simulink model "esp32p4_foc"  (R2025b)
settings: Solver=FixedStepDiscrete  StartTime=0.0  StopTime=sim_end_s  FixedStep=Ts_plant  RelTol=1e-3
model workspace: external: MATLAB File esp32p4_foc_data.m (data not in the file)
values from neighbouring files (symbols this model uses):
  adc_bits = 12    [esp32p4_foc_data.m]
  adc_range_mV = 3100    [esp32p4_foc_data.m]
  alpha_w = 0.05    [esp32p4_foc_data.m]
  B_m = B_rotor + B_load    (= 1.07e-06)    [esp32p4_foc_data.m]
  b_u_mV = 1680    [esp32p4_foc_data.m]
  b_v_mV = 1680    [esp32p4_foc_data.m]
  ctrl_dt_max_s = 0.05    [esp32p4_foc_data.m]
  duty_mid = 0.5    [esp32p4_foc_data.m]
  enc_bits = 12    [esp32p4_foc_data.m]
  enc_dt_max_us = 20000    [esp32p4_foc_data.m]
  enc_dt_min_us = 100    [esp32p4_foc_data.m]
  enc_fail_decay = 0.9    [esp32p4_foc_data.m]
  enc_ok = 1    [esp32p4_foc_data.m]
  f_closed_max_Hz = 60    [esp32p4_foc_data.m]
  f_console_max_Hz = 80    [esp32p4_foc_data.m]
  I_console_max_mA = 1800    [esp32p4_foc_data.m]
  id_target_mA = 0    [esp32p4_foc_data.m]
  Imax = 200    [esp32p4_foc_data.m]
  J_m = J_rotor + J_load    (= 5e-07)    [esp32p4_foc_data.m]
  Ki_i = 8.0e-4    (= 0.0008)    [esp32p4_foc_data.m]
  Ki_w = 200    [esp32p4_foc_data.m]
  Kp_i = 2.5e-4    (= 0.00025)    [esp32p4_foc_data.m]
  Kp_w = 27    [esp32p4_foc_data.m]
  L_d = 2.58e-3    (= 0.00258)    [esp32p4_foc_data.m]
  L_q = L_d    (= 0.00258)    [esp32p4_foc_data.m]
  load_Nm = 0.002    [esp32p4_foc_data.m]
  mod_limit = 0.40    (= 0.4)    [esp32p4_foc_data.m]
  motor_x0 = [0; 0; 0; 0]    [esp32p4_foc_data.m]
  ocp_disable_s = 0.020    (= 0.02)    [esp32p4_foc_data.m]
  ocp_limit_mA = 1500    [esp32p4_foc_data.m]
  ocp_samples = 150    [esp32p4_foc_data.m]
  p_pairs = 7    [esp32p4_foc_data.m]
  psi_pm = Ke_LL_rms_per_krpm * sqrt(2/3) / (p_pairs * (1000*2*pi/60))    [esp32p4_foc_data.m]
  pwm_bits = 10    [esp32p4_foc_data.m]
  pwm_Hz = 20000    [esp32p4_foc_data.m]
  pwm_switching = 0    [esp32p4_foc_data.m]
  R_s = 18.76    [esp32p4_foc_data.m]
  R_shunt = 0.015    [esp32p4_foc_data.m]
  s_enc = 1    [esp32p4_foc_data.m]
  sense_gain = 50    [esp32p4_foc_data.m]
  sense_sign = -1    [esp32p4_foc_data.m]
  sense_wiring_sign = -1    [esp32p4_foc_data.m]
  start_Hz = 0    [esp32p4_foc_data.m]
  start_load_Nm = 0    [esp32p4_foc_data.m]
  step_load_s = 1.25    [esp32p4_foc_data.m]
  step_speed_s = 0.10    (= 0.1)    [esp32p4_foc_data.m]
  target_Hz = 8    [esp32p4_foc_data.m]
  theta_off = 0    [esp32p4_foc_data.m]
  torque_sign = 1    [esp32p4_foc_data.m]
  Ts_ctrl = 1e-3    (= 0.001)    [esp32p4_foc_data.m]
  Ts_plant = 1e-5    (= 1e-05)    [esp32p4_foc_data.m]
  unipolar_threshold_mV = 300    [esp32p4_foc_data.m]
  V_dc = 12    [esp32p4_foc_data.m]
Description:
  | ESP32-P4 M2: cascaded electrical speed and dq current control.
  | Firmware BassttElSevic/esp32p4-foc @ c20fad4. Starts calibrated in RUN.
  | Illustrative plant parameters are in the Model Workspace. Open the FOC subsystem to inspect the loops.
settings Model: Creator=29113  LastModifiedBy=29113
settings DataIOCC: SaveOutput=off  SaveTime=off

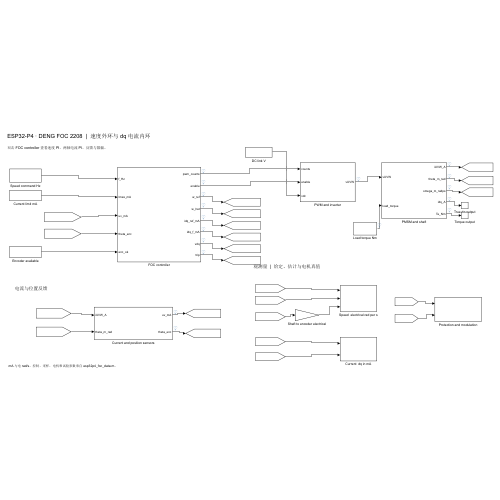
[thumbnail: Simulink's stored preview of the top-level diagram]
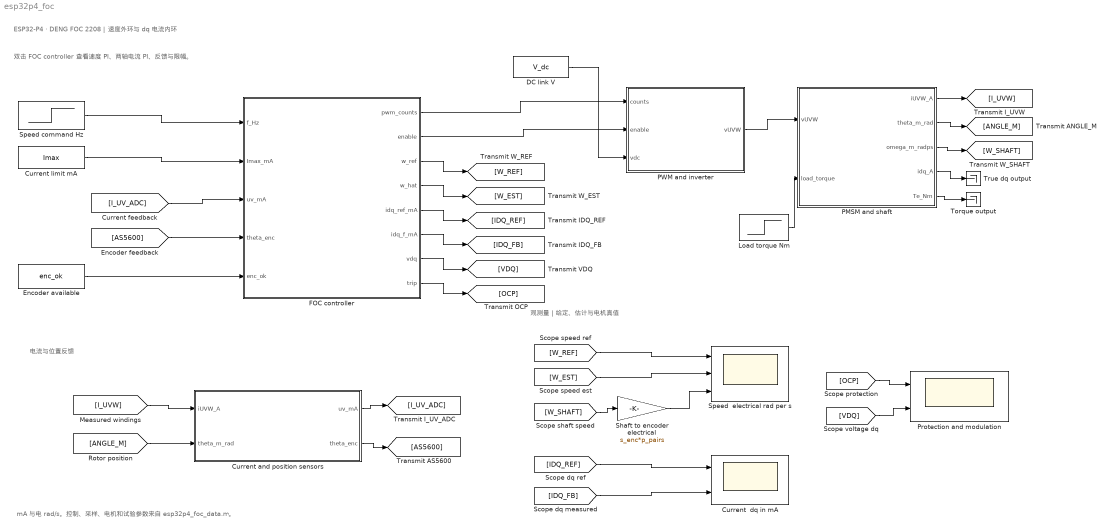
== system esp32p4_foc ==
  note: ESP32-P4 · DENG FOC 2208 | 速度外环与 dq 电流内环
  note: 双击 FOC controller 查看速度 PI、两轴电流 PI、反馈与限幅。
  note: 电流与位置反馈
  note: 观测量 | 给定、估计与电机真值
  note: mA 与电 rad/s。控制、采样、电机和试验参数来自 esp32p4_foc_data.m。
  Current  dq in mA : Scope  NumInputPorts=2
  Current and position sensors : Subsystem
  Current limit mA : Constant  Value=Imax  SampleTime=Ts_ctrl
  DC link V : Constant  Value=V_dc  SampleTime=Ts_plant
  Encoder available : Constant  Value=enc_ok  SampleTime=Ts_ctrl
  FOC controller : Subsystem
  Load torque Nm : Step  Time=step_load_s  Before=start_load_Nm  After=load_Nm  SampleTime=Ts_plant
  PMSM and shaft : Subsystem
  PWM and inverter : Subsystem
  Protection and modulation : Scope  NumInputPorts=2
  Shaft to encoder electrical : Gain  Gain=s_enc*p_pairs
  Speed  electrical rad per s : Scope  NumInputPorts=3
  Speed command Hz : Step  Time=step_speed_s  Before=start_Hz  After=target_Hz  SampleTime=Ts_ctrl
  Torque output : Terminator
  True dq output : Terminator
  wires:
  Speed command Hz/1 -> FOC controller/1(f_Hz)
  Current limit mA/1 -> FOC controller/2(Imax_mA)
  Encoder available/1 -> FOC controller/5(enc_ok)
  FOC controller/1(pwm_counts) -> PWM and inverter/1(counts)
  FOC controller/2(enable) -> PWM and inverter/2(enable)
  DC link V/1 -> PWM and inverter/3(vdc)
  PWM and inverter/1(vUVW) -> PMSM and shaft/1(vUVW)
  Load torque Nm/1 -> PMSM and shaft/2(load_torque)
  PMSM and shaft/1(iUVW_A) -> [I_UVW]
  PMSM and shaft/2(theta_m_rad) -> [ANGLE_M]
  [I_UVW] -> Current and position sensors/1(iUVW_A)
  [ANGLE_M] -> Current and position sensors/2(theta_m_rad)
  Current and position sensors/1(uv_mA) -> [I_UV_ADC]
  Current and position sensors/2(theta_enc) -> [AS5600]
  [I_UV_ADC] -> FOC controller/3(uv_mA)
  [AS5600] -> FOC controller/4(theta_enc)
  FOC controller/3(w_ref) -> [W_REF]
  FOC controller/4(w_hat) -> [W_EST]
  FOC controller/5(idq_ref_mA) -> [IDQ_REF]
  FOC controller/6(idq_f_mA) -> [IDQ_FB]
  FOC controller/7(vdq) -> [VDQ]
  FOC controller/8(trip) -> [OCP]
  PMSM and shaft/3(omega_m_radps) -> [W_SHAFT]
  PMSM and shaft/4(idq_A) -> True dq output/1
  PMSM and shaft/5(Te_Nm) -> Torque output/1
  [W_REF] -> Speed  electrical rad per s/1
  [W_EST] -> Speed  electrical rad per s/2
  [W_SHAFT] -> Shaft to encoder electrical/1
  Shaft to encoder electrical/1 -> Speed  electrical rad per s/3
  [IDQ_REF] -> Current  dq in mA/1
  [IDQ_FB] -> Current  dq in mA/2
  [OCP] -> Protection and modulation/1
  [VDQ] -> Protection and modulation/2

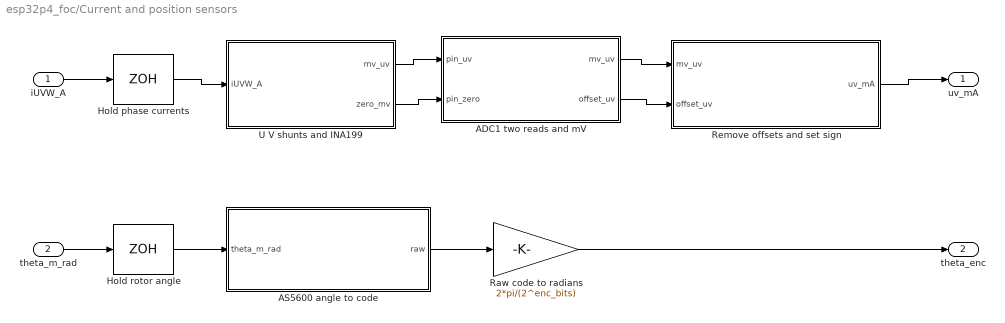
== system esp32p4_foc/Current and position sensors ==
  iUVW_A : Inport
  theta_m_rad : Inport  Port=2
  ADC1 two reads and mV : MATLAB Function  TreatAsAtomicUnit=on
  AS5600 angle to code : MATLAB Function  TreatAsAtomicUnit=on
  Hold phase currents : ZeroOrderHold  SampleTime=Ts_ctrl
  Hold rotor angle : ZeroOrderHold  SampleTime=Ts_ctrl
  Raw code to radians : Gain  Gain=2*pi/(2^enc_bits)
  Remove offsets and set sign : MATLAB Function  TreatAsAtomicUnit=on
  U V shunts and INA199 : MATLAB Function  TreatAsAtomicUnit=on
  uv_mA : Outport
  theta_enc : Outport  Port=2
  wires:
  iUVW_A/1 -> Hold phase currents/1
  Hold phase currents/1 -> U V shunts and INA199/1(iUVW_A)
  U V shunts and INA199/1(mv_uv) -> ADC1 two reads and mV/1(pin_uv)
  U V shunts and INA199/2(zero_mv) -> ADC1 two reads and mV/2(pin_zero)
  ADC1 two reads and mV/1(mv_uv) -> Remove offsets and set sign/1(mv_uv)
  ADC1 two reads and mV/2(offset_uv) -> Remove offsets and set sign/2(offset_uv)
  Remove offsets and set sign/1(uv_mA) -> uv_mA/1
  theta_m_rad/1 -> Hold rotor angle/1
  Hold rotor angle/1 -> AS5600 angle to code/1(theta_m_rad)
  AS5600 angle to code/1(raw) -> Raw code to radians/1
  Raw code to radians/1 -> theta_enc/1

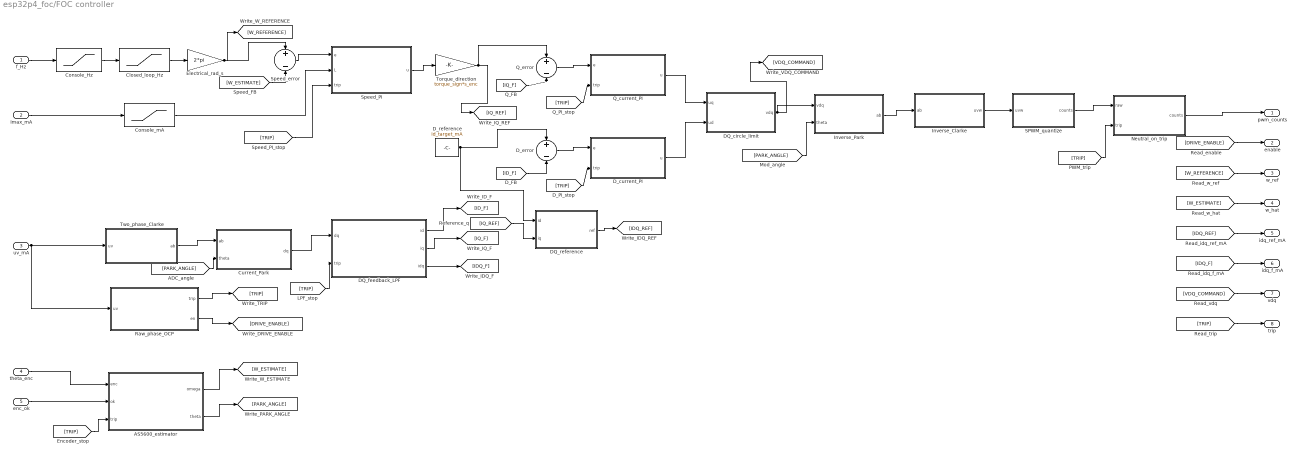
== system esp32p4_foc/FOC controller ==
  f_Hz : Inport
  Imax_mA : Inport  Port=2
  uv_mA : Inport  Port=3
  theta_enc : Inport  Port=4
  enc_ok : Inport  Port=5
  AS5600_estimator : MATLAB Function  TreatAsAtomicUnit=on
  Closed_loop_Hz : Saturate  UpperLimit=f_closed_max_Hz  LowerLimit=-f_closed_max_Hz
  Console_Hz : Saturate  UpperLimit=f_console_max_Hz  LowerLimit=-f_console_max_Hz
  Console_mA : Saturate  UpperLimit=I_console_max_mA  LowerLimit=-I_console_max_mA
  Current_Park : MATLAB Function  TreatAsAtomicUnit=on
  DQ_circle_limit : MATLAB Function  TreatAsAtomicUnit=on
  DQ_feedback_LPF : MATLAB Function  TreatAsAtomicUnit=on
  DQ_reference : MATLAB Function  TreatAsAtomicUnit=on
  D_current_PI : MATLAB Function  TreatAsAtomicUnit=on
  D_error : Sum  Inputs=+-
  D_reference : Constant  Value=id_target_mA
  Electrical_rad_s : Gain  Gain=2*pi
  Inverse_Clarke : MATLAB Function  TreatAsAtomicUnit=on
  Inverse_Park : MATLAB Function  TreatAsAtomicUnit=on
  Neutral_on_trip : MATLAB Function  TreatAsAtomicUnit=on
  Q_current_PI : MATLAB Function  TreatAsAtomicUnit=on
  Q_error : Sum  Inputs=+-
  Raw_phase_OCP : MATLAB Function  TreatAsAtomicUnit=on
  SPWM_quantize : MATLAB Function  TreatAsAtomicUnit=on
  Speed_PI : MATLAB Function  TreatAsAtomicUnit=on
  Speed_error : Sum  Inputs=+-
  Torque_direction : Gain  Gain=torque_sign*s_enc
  Two_phase_Clarke : MATLAB Function  TreatAsAtomicUnit=on
  pwm_counts : Outport
  enable : Outport  Port=2
  w_ref : Outport  Port=3
  w_hat : Outport  Port=4
  idq_ref_mA : Outport  Port=5
  idq_f_mA : Outport  Port=6
  vdq : Outport  Port=7
  trip : Outport  Port=8
  wires:
  Electrical_rad_s/1 -> [W_REFERENCE], Speed_error/1
  DQ_circle_limit/1(vdq) -> [VDQ_COMMAND], Inverse_Park/1(vdq)
  Torque_direction/1 -> [IQ_REF], Q_error/1
  DQ_feedback_LPF/1(id) -> [ID_F]
  DQ_feedback_LPF/2(iq) -> [IQ_F]
  DQ_feedback_LPF/3(idq) -> [IDQ_F]
  Raw_phase_OCP/1(trip) -> [TRIP]
  Raw_phase_OCP/2(en) -> [DRIVE_ENABLE]
  AS5600_estimator/1(omega) -> [W_ESTIMATE]
  AS5600_estimator/2(theta) -> [PARK_ANGLE]
  DQ_reference/1(ref) -> [IDQ_REF]
  [W_ESTIMATE] -> Speed_error/2
  [TRIP] -> Speed_PI/3(trip)
  [IQ_F] -> Q_error/2
  [ID_F] -> D_error/2
  [TRIP] -> Q_current_PI/2(trip)
  [TRIP] -> D_current_PI/2(trip)
  [PARK_ANGLE] -> Inverse_Park/2(theta)
  [TRIP] -> Neutral_on_trip/2(trip)
  [PARK_ANGLE] -> Current_Park/2(theta)
  [TRIP] -> DQ_feedback_LPF/2(trip)
  [TRIP] -> AS5600_estimator/3(trip)
  [IQ_REF] -> DQ_reference/2(iq)
  f_Hz/1 -> Console_Hz/1
  Console_Hz/1 -> Closed_loop_Hz/1
  Closed_loop_Hz/1 -> Electrical_rad_s/1
  Speed_error/1 -> Speed_PI/1(e)
  Imax_mA/1 -> Console_mA/1
  Console_mA/1 -> Speed_PI/2(L)
  Speed_PI/1(u) -> Torque_direction/1
  Q_error/1 -> Q_current_PI/1(e)
  D_reference/1 -> D_error/1, DQ_reference/1(id)
  D_error/1 -> D_current_PI/1(e)
  Q_current_PI/1(u) -> DQ_circle_limit/1(uq)
  D_current_PI/1(u) -> DQ_circle_limit/2(ud)
  Inverse_Park/1(ab) -> Inverse_Clarke/1(ab)
  Inverse_Clarke/1(uvw) -> SPWM_quantize/1(uvw)
  SPWM_quantize/1(counts) -> Neutral_on_trip/1(raw)
  uv_mA/1 -> Two_phase_Clarke/1(uv), Raw_phase_OCP/1(uv)
  Two_phase_Clarke/1(ab) -> Current_Park/1(ab)
  Current_Park/1(dq) -> DQ_feedback_LPF/1(dq)
  theta_enc/1 -> AS5600_estimator/1(enc)
  enc_ok/1 -> AS5600_estimator/2(ok)
  Neutral_on_trip/1(counts) -> pwm_counts/1
  [DRIVE_ENABLE] -> enable/1
  [W_REFERENCE] -> w_ref/1
  [W_ESTIMATE] -> w_hat/1
  [IDQ_REF] -> idq_ref_mA/1
  [IDQ_F] -> idq_f_mA/1
  [VDQ_COMMAND] -> vdq/1
  [TRIP] -> trip/1

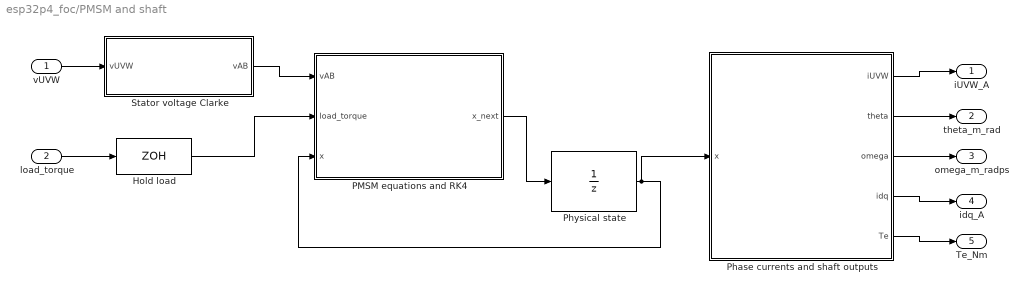
== system esp32p4_foc/PMSM and shaft ==
  vUVW : Inport
  load_torque : Inport  Port=2
  Hold load : ZeroOrderHold  SampleTime=Ts_plant
  PMSM equations and RK4 : MATLAB Function  TreatAsAtomicUnit=on
  Phase currents and shaft outputs : MATLAB Function  TreatAsAtomicUnit=on
  Physical state : UnitDelay  InitialCondition=motor_x0  SampleTime=Ts_plant  HasFrameUpgradeWarning=on
  Stator voltage Clarke : MATLAB Function  TreatAsAtomicUnit=on
  iUVW_A : Outport
  theta_m_rad : Outport  Port=2
  omega_m_radps : Outport  Port=3
  idq_A : Outport  Port=4
  Te_Nm : Outport  Port=5
  wires:
  Phase currents and shaft outputs/1(iUVW) -> iUVW_A/1
  Phase currents and shaft outputs/2(theta) -> theta_m_rad/1
  Phase currents and shaft outputs/3(omega) -> omega_m_radps/1
  Phase currents and shaft outputs/4(idq) -> idq_A/1
  Phase currents and shaft outputs/5(Te) -> Te_Nm/1
  vUVW/1 -> Stator voltage Clarke/1(vUVW)
  Stator voltage Clarke/1(vAB) -> PMSM equations and RK4/1(vAB)
  load_torque/1 -> Hold load/1
  Hold load/1 -> PMSM equations and RK4/2(load_torque)
  Physical state/1 -> PMSM equations and RK4/3(x), Phase currents and shaft outputs/1(x)
  PMSM equations and RK4/1(x_next) -> Physical state/1

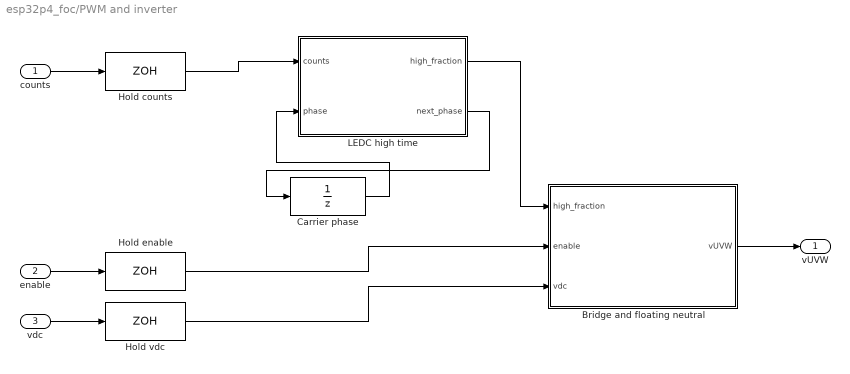
== system esp32p4_foc/PWM and inverter ==
  counts : Inport
  enable : Inport  Port=2
  vdc : Inport  Port=3
  Bridge and floating neutral : MATLAB Function  TreatAsAtomicUnit=on
  Carrier phase : UnitDelay  SampleTime=Ts_plant  HasFrameUpgradeWarning=on
  Hold counts : ZeroOrderHold  SampleTime=Ts_plant
  Hold enable : ZeroOrderHold  SampleTime=Ts_plant
  Hold vdc : ZeroOrderHold  SampleTime=Ts_plant
  LEDC high time : MATLAB Function  TreatAsAtomicUnit=on
  vUVW : Outport
  wires:
  counts/1 -> Hold counts/1
  enable/1 -> Hold enable/1
  vdc/1 -> Hold vdc/1
  Hold counts/1 -> LEDC high time/1(counts)
  Carrier phase/1 -> LEDC high time/2(phase)
  LEDC high time/2(next_phase) -> Carrier phase/1
  LEDC high time/1(high_fraction) -> Bridge and floating neutral/1(high_fraction)
  Hold enable/1 -> Bridge and floating neutral/2(enable)
  Hold vdc/1 -> Bridge and floating neutral/3(vdc)
  Bridge and floating neutral/1(vUVW) -> vUVW/1

== matlab function esp32p4_foc/FOC controller/Two_phase_Clarke ==
  data: uv input; ab output
function ab = fcn(uv)
ab = [uv(1);(uv(1)+2*uv(2))/sqrt(3)];
end

== matlab function esp32p4_foc/FOC controller/Current_Park ==
  data: ab input; dq output; theta input
function dq = fcn(ab,theta)
c = cos(theta); s = sin(theta);
dq = [ab(1)*c+ab(2)*s;-ab(1)*s+ab(2)*c];
end

== matlab function esp32p4_foc/FOC controller/DQ_feedback_LPF ==
  data: dq input; id output; trip input; iq output; idq output; alpha_i parameter
function [id,iq,idq] = fcn(dq,trip, alpha_i)
persistent filtered
if isempty(filtered), filtered = zeros(2,1); end
if trip == 0
    filtered = filtered + alpha_i*(dq-filtered);
end
idq = filtered; id = filtered(1); iq = filtered(2);
end

== matlab function esp32p4_foc/FOC controller/Raw_phase_OCP ==
  data: uv input; trip output; en output; Ts_ctrl parameter; ocp_limit_mA parameter; ocp_samples parameter; ocp_disable_s parameter
function [trip,en] = fcn(uv, Ts_ctrl, ocp_limit_mA, ocp_samples, ocp_disable_s)
persistent hits tripped elapsedTicks
if isempty(hits), hits = 0; tripped = false; elapsedTicks = 0; end
if tripped
    elapsedTicks = elapsedTicks+1;
else
    peak = max([abs(uv(1));abs(uv(2));abs(-uv(1)-uv(2))]);
    if peak > ocp_limit_mA, hits = hits+1; else, hits = 0; end
    if hits >= ocp_samples, tripped = true; elapsedTicks = 0; end
end
trip = double(tripped);
en = double(~tripped || round(elapsedTicks*Ts_ctrl*1e6) < round(ocp_disable_s*1e6));
end

== matlab function esp32p4_foc/FOC controller/AS5600_estimator ==
  data: enc input; omega output; ok input; trip input; theta output; Ts_ctrl parameter; p_pairs parameter; s_enc parameter; theta_off parameter; enc_dt_min_us parameter; enc_dt_max_us parameter; alpha_w parameter; enc_fail_decay parameter; ctrl_dt_max_s parameter
function [omega,theta] = fcn(enc,ok,trip, Ts_ctrl, p_pairs, s_enc, theta_off, enc_dt_min_us, enc_dt_max_us, alpha_w, enc_fail_decay, ctrl_dt_max_s)
persistent previous estimate ticks initialized
if isempty(ticks)
    previous = 0; estimate = 0; ticks = 0; initialized = false;
end
if trip == 0
    ticks = ticks+1;
    if ok ~= 0
        delta = enc-previous;
        if delta > pi, delta = delta-2*pi; end
        if delta < -pi, delta = delta+2*pi; end
        dt_us = round(ticks*Ts_ctrl*1e6);
        if initialized && dt_us > enc_dt_min_us && dt_us < enc_dt_max_us
            raw = p_pairs*delta/(dt_us*1e-6);
            estimate = estimate + alpha_w*(raw-estimate);
        end
        previous = enc; initialized = true; ticks = 0;
    else
        estimate = enc_fail_decay*estimate;
    end
end
omega = estimate;
theta = mod(mod(s_enc*p_pairs*previous+theta_off,2*pi)+omega*min(ctrl_dt_max_s,max(0,Ts_ctrl)),2*pi);
end

== matlab function esp32p4_foc/FOC controller/DQ_reference ==
  data: id input; ref output; iq input
function ref = fcn(id,iq)
ref = [id;iq];
end

== matlab function esp32p4_foc/PWM and inverter/LEDC high time ==
  data: counts input; high_fraction output; phase input; next_phase output; Ts_plant parameter; pwm_switching parameter; pwm_Hz parameter; pwm_bits parameter
function [high_fraction, next_phase] = pwm_interval(counts, phase, Ts_plant, pwm_switching, pwm_Hz, pwm_bits)
%#codegen
% The hardware counter has 2^pwm_bits states, with a high fraction of N/levels.
% The interval starts at the stored leading-edge carrier phase.
levels = 2^pwm_bits;
periods = pwm_Hz * Ts_plant;
stop = phase + periods;
next_phase = mod(stop,1);
high_fraction = zeros(3,1);
for k = 1:3
    duty = min(levels-1,max(0,round(counts(k)))) / levels;
    if pwm_switching ~= 0
        % Integral of the rectangular pulse train, in carrier periods.
        start_area = min(phase,duty);
        stop_area = floor(stop)*duty + min(mod(stop,1),duty);
        high_fraction(k) = min(1,max(0,(stop_area-start_area)/periods));
    else
        high_fraction(k) = duty;
    end
end
end

== matlab function esp32p4_foc/PWM and inverter/Bridge and floating neutral ==
  data: high_fraction input; vUVW output; enable input; vdc input
function vUVW = bridge_voltage(high_fraction, enable, vdc)
%#codegen
% An ideal two-level bridge feeding a balanced three-wire star.
vUVW = zeros(3,1);
if enable ~= 0
    v_pole = vdc * high_fraction;
    v_neutral = (v_pole(1) + v_pole(2) + v_pole(3)) / 3;
    vUVW = v_pole - v_neutral;
end
% Disabled approximation: equal pole potentials, zero line-line voltages.
end

== matlab function esp32p4_foc/PMSM and shaft/Stator voltage Clarke ==
  data: vUVW input; vAB output
function vAB = stator_voltage(vUVW)
%#codegen
% Amplitude-invariant Clarke transform; common mode cancels.
vAB = [(2*vUVW(1)-vUVW(2)-vUVW(3))/3; (vUVW(2)-vUVW(3))/sqrt(3)];
end

== matlab function esp32p4_foc/FOC controller/Q_current_PI ==
  data: e input; u output; trip input; Ts_ctrl parameter; Kp_i parameter; Ki_i parameter; mod_limit parameter; ctrl_dt_max_s parameter
function u = fcn(e,trip, Ts_ctrl, Kp_i, Ki_i, mod_limit, ctrl_dt_max_s)
persistent x held
if isempty(x), x = 0; held = 0; end
L = mod_limit;
if trip ~= 0, u = held; return; end
b = x + Kp_i*e;
delta = Ki_i*e*min(ctrl_dt_max_s,max(0,Ts_ctrl));
if b > L
    u = L; if e < 0, x = x+delta; end
elseif b < -L
    u = -L; if e > 0, x = x+delta; end
else
    u = b; x = x+delta;
end
if x > L, x = L; end
if x < -L, x = -L; end
held = u;
end

== matlab function esp32p4_foc/PMSM and shaft/PMSM equations and RK4 ==
  data: vAB input; x_next output; load_torque input; x input; Ts_plant parameter; p_pairs parameter; R_s parameter; L_d parameter; L_q parameter; psi_pm parameter; J_m parameter; B_m parameter
function x_next = advance_pmsm(vAB, load_torque, x, Ts_plant, p_pairs, R_s, L_d, L_q, psi_pm, J_m, B_m)
%#codegen
% x = [id (A); iq (A); mechanical angle (rad); mechanical speed (rad/s)].
% Hold stationary-frame voltage and load over the integration interval.
h = Ts_plant;
k1 = derivative(x,vAB,load_torque,p_pairs,R_s,L_d,L_q,psi_pm,J_m,B_m);
k2 = derivative(x+h*k1/2,vAB,load_torque,p_pairs,R_s,L_d,L_q,psi_pm,J_m,B_m);
k3 = derivative(x+h*k2/2,vAB,load_torque,p_pairs,R_s,L_d,L_q,psi_pm,J_m,B_m);
k4 = derivative(x+h*k3,vAB,load_torque,p_pairs,R_s,L_d,L_q,psi_pm,J_m,B_m);
x_next = x + (h/6)*(k1+2*k2+2*k3+k4);
end

function dx = derivative(x,vAB,load_torque,p,R,Ld,Lq,psi,J,B)
id = x(1); iq = x(2); theta = x(3); omega = x(4);
ct = cos(p*theta); st = sin(p*theta);
vd =  ct*vAB(1) + st*vAB(2);
vq = -st*vAB(1) + ct*vAB(2);
we = p*omega;
did = (vd - R*id + we*Lq*iq)/Ld;
diq = (vq - R*iq - we*(Ld*id + psi))/Lq;
Te = 1.5*p*(psi + (Ld-Lq)*id)*iq;
dx = [did; diq; omega; (Te - load_torque - B*omega)/J];
end

== matlab function esp32p4_foc/PMSM and shaft/Phase currents and shaft outputs ==
  data: x input; iUVW output; theta output; omega output; idq output; Te output; p_pairs parameter; L_d parameter; L_q parameter; psi_pm parameter
function [iUVW,theta,omega,idq,Te] = outputs(x, p_pairs, L_d, L_q, psi_pm)
%#codegen
id = x(1); iq = x(2); theta = x(3); omega = x(4);
ct = cos(p_pairs*theta); st = sin(p_pairs*theta);
i_alpha = ct*id - st*iq;
i_beta = st*id + ct*iq;
iUVW = [i_alpha; -.5*i_alpha + sqrt(3)*.5*i_beta; -.5*i_alpha - sqrt(3)*.5*i_beta];
idq = [id; iq];
Te = 1.5*p_pairs*(psi_pm+(L_d-L_q)*id)*iq;
end

== matlab function esp32p4_foc/Current and position sensors/U V shunts and INA199 ==
  data: iUVW_A input; mv_uv output; zero_mv output; b_u_mV parameter; b_v_mV parameter; R_shunt parameter; sense_gain parameter; sense_wiring_sign parameter
function [mv_uv, zero_mv] = sense(iUVW_A, b_u_mV, b_v_mV, R_shunt, sense_gain, sense_wiring_sign)
% The physical shunt polarity is independent of the software sign correction.
zero_mv = [b_u_mV; b_v_mV];
amps_uv = [iUVW_A(1); iUVW_A(2)];
mv_uv = zero_mv + sense_wiring_sign * (1000 * R_shunt * sense_gain) * amps_uv;
end

== matlab function esp32p4_foc/Current and position sensors/ADC1 two reads and mV ==
  data: pin_uv input; mv_uv output; pin_zero input; offset_uv output; adc_bits parameter; adc_range_mV parameter
function [mv_uv, offset_uv] = adc(pin_uv, pin_zero, adc_bits, adc_range_mV)
% Running samples and the stationary zero calibration use the same ADC model.
last_code = 2^adc_bits - 1;
mv_uv = adc_read_mv(pin_uv, last_code, adc_range_mV);
offset_uv = adc_read_mv(pin_zero, last_code, adc_range_mV);
end
function mv = adc_read_mv(pin_mv, last_code, range_mv)
% The two one-shot reads see the same held voltage. Their integer mean is raw.
clipped_mv = min(max(pin_mv, 0), range_mv);
raw = floor(clipped_mv * (last_code/range_mv) + 0.5);
% main.c:525, without a chip-specific calibration curve.
mv = floor((raw * range_mv) / last_code);
end

== matlab function esp32p4_foc/Current and position sensors/Remove offsets and set sign ==
  data: mv_uv input; uv_mA output; offset_uv input; R_shunt parameter; sense_gain parameter; sense_sign parameter; unipolar_threshold_mV parameter
function uv_mA = convert(mv_uv, offset_uv, R_shunt, sense_gain, sense_sign, unipolar_threshold_mV)
% A stationary, disabled motor gives identical readings throughout zero calibration.
delta_mv = mv_uv - offset_uv;
if all(offset_uv < unipolar_threshold_mV)
    delta_mv = max(delta_mv, 0);
end
uv_mA = sense_sign * delta_mv / (R_shunt * sense_gain);
end

== matlab function esp32p4_foc/Current and position sensors/AS5600 angle to code ==
  data: theta_m_rad input; raw output; s_enc parameter; p_pairs parameter; theta_off parameter; enc_bits parameter
function raw = encoder(theta_m_rad, s_enc, p_pairs, theta_off, enc_bits)
% Sensor mounting is the inverse of the calibrated mech_to_elec relationship.
angle_rad = mod(s_enc * (theta_m_rad - theta_off / p_pairs), 2*pi);
% Select the angular bin that contains the actual mechanical angle.
bins = 2^enc_bits;
raw = min(bins-1, floor(angle_rad * (bins/(2*pi))));
end

== matlab function esp32p4_foc/FOC controller/Speed_PI ==
  data: e input; u output; L input; trip input; Ts_ctrl parameter; Kp_w parameter; Ki_w parameter; ctrl_dt_max_s parameter
function u = fcn(e,L,trip, Ts_ctrl, Kp_w, Ki_w, ctrl_dt_max_s)
persistent x held
if isempty(x), x = 0; held = 0; end
% L is the signed console argument after command saturation.
if trip ~= 0, u = held; return; end
b = x + Kp_w*e;
delta = Ki_w*e*min(ctrl_dt_max_s,max(0,Ts_ctrl));
if b > L
    u = L; if e < 0, x = x+delta; end
elseif b < -L
    u = -L; if e > 0, x = x+delta; end
else
    u = b; x = x+delta;
end
if x > L, x = L; end
if x < -L, x = -L; end
held = u;
end

== matlab function esp32p4_foc/FOC controller/D_current_PI ==
  data: e input; u output; trip input; Ts_ctrl parameter; Kp_i parameter; Ki_i parameter; mod_limit parameter; ctrl_dt_max_s parameter
function u = fcn(e,trip, Ts_ctrl, Kp_i, Ki_i, mod_limit, ctrl_dt_max_s)
persistent x held
if isempty(x), x = 0; held = 0; end
L = mod_limit;
if trip ~= 0, u = held; return; end
b = x + Kp_i*e;
delta = Ki_i*e*min(ctrl_dt_max_s,max(0,Ts_ctrl));
if b > L
    u = L; if e < 0, x = x+delta; end
elseif b < -L
    u = -L; if e > 0, x = x+delta; end
else
    u = b; x = x+delta;
end
if x > L, x = L; end
if x < -L, x = -L; end
held = u;
end

== matlab function esp32p4_foc/FOC controller/DQ_circle_limit ==
  data: uq input; vdq output; ud input; mod_limit parameter
function vdq = fcn(uq,ud, mod_limit)
r = sqrt(ud*ud + uq*uq);
vdq = [ud;uq];
if r > mod_limit
    vdq = (mod_limit/r)*vdq;
end
end

== matlab function esp32p4_foc/FOC controller/Inverse_Park ==
  data: vdq input; ab output; theta input
function ab = fcn(vdq,theta)
c = cos(theta); s = sin(theta);
ab = [vdq(1)*c-vdq(2)*s;vdq(1)*s+vdq(2)*c];
end

== matlab function esp32p4_foc/FOC controller/Inverse_Clarke ==
  data: ab input; uvw output
function uvw = fcn(ab)
a = ab(1); b = ab(2);
uvw = [a; -0.5*a+0.5*sqrt(3)*b; -0.5*a-0.5*sqrt(3)*b];
end

== matlab function esp32p4_foc/FOC controller/SPWM_quantize ==
  data: uvw input; counts output; pwm_bits parameter; duty_mid parameter
function counts = fcn(uvw, pwm_bits, duty_mid)
counts = floor((2^pwm_bits-1)*max(0,min(1,duty_mid+uvw))+0.5);
end

== matlab function esp32p4_foc/FOC controller/Neutral_on_trip ==
  data: raw input; counts output; trip input; pwm_bits parameter; duty_mid parameter
function counts = fcn(raw,trip, pwm_bits, duty_mid)
if trip ~= 0
    counts = ones(3,1)*floor((2^pwm_bits-1)*duty_mid+0.5);
else
    counts = raw;
end
end
